simulink model "FMT_X4_ControlAllocation"  (R2026b)
settings: Solver=FixedStepDiscrete  StopTime=2
settings Model: DataDictionary=Flight_Parameters.sldd  Creator=26718  LastModifiedBy=26718

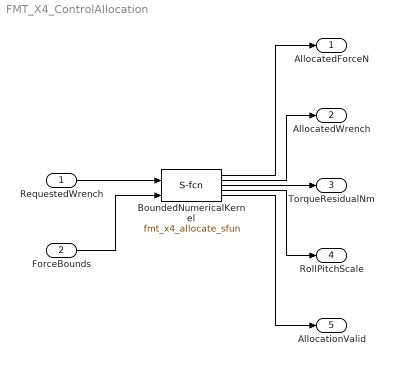
== system FMT_X4_ControlAllocation ==
  RequestedWrench : Inport  OutDataTypeStr=double  PortDimensions=4
  ForceBounds : Inport  Port=2  OutDataTypeStr=double  PortDimensions=8
  BoundedNumericalKernel : S-Function  FunctionName=fmt_x4_allocate_sfun  Parameters=AllocationGeometry  SFunctionDeploymentMode=off  EnableBusSupport=off
  AllocatedForceN : Outport
  AllocatedWrench : Outport  Port=2
  TorqueResidualNm : Outport  Port=3
  RollPitchScale : Outport  Port=4
  AllocationValid : Outport  Port=5
  wires:
  BoundedNumericalKernel/5 -> AllocationValid/1
  BoundedNumericalKernel/4 -> RollPitchScale/1
  BoundedNumericalKernel/3 -> TorqueResidualNm/1
  BoundedNumericalKernel/2 -> AllocatedWrench/1
  BoundedNumericalKernel/1 -> AllocatedForceN/1
  ForceBounds/1 -> BoundedNumericalKernel/2
  RequestedWrench/1 -> BoundedNumericalKernel/1
